simulink model "PIDControl"  (R2024b)
settings: Solver=VariableStepAuto  StartTime=0.0  StopTime=10.0  RelTol=1e-3
settings Model: Creator=mfussi  LastModifiedBy=mfussi

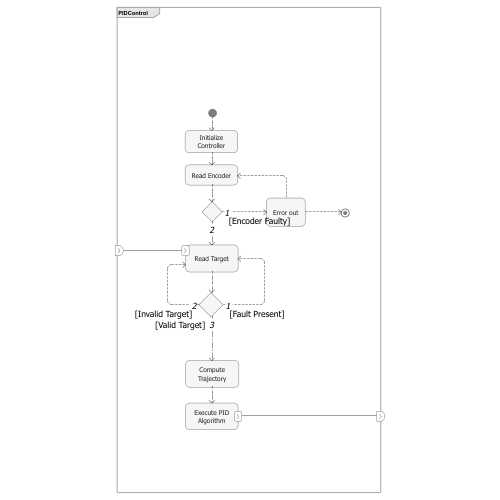
[thumbnail: Simulink's stored preview of the top-level diagram]
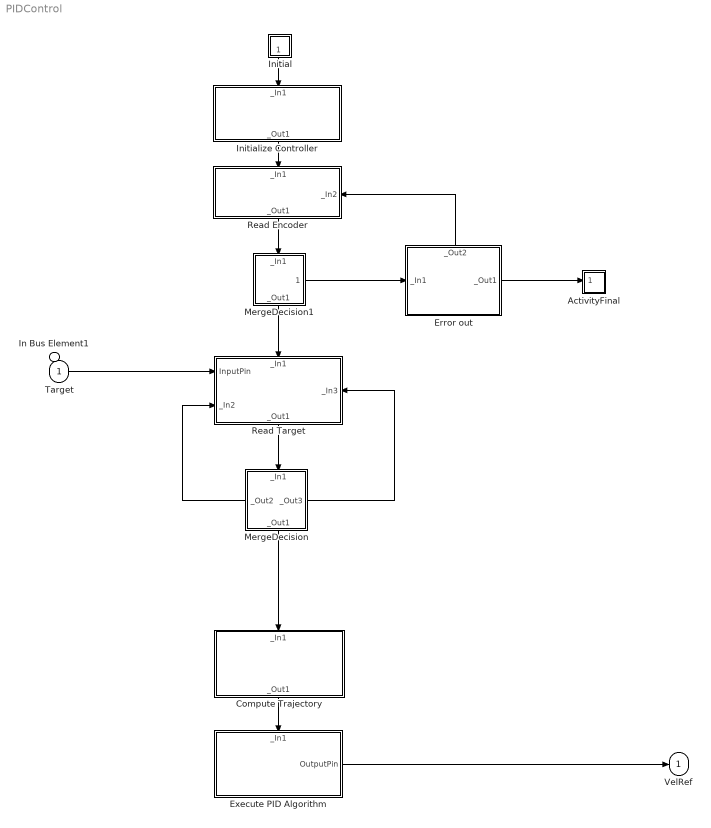
== system PIDControl ==
  Target : Inport
  In Bus Element1 : Inport  Port=2  PortName=Mode Selector
  ActivityFinal : Subsystem
      settings: CopyFcn=set_param(gcbh,'LinkStatus','none');  PortSchema="{\"entries\":[{\"content\":{\"sides\":[{\"content\":{\"connectorIds\":[\"In1\"]},\"type\":\"ConnectorPlacement.EquallySpacedRectSide\",\"uuid\":\"678327c4-9999-46ea-b1a4-4ad8eb3b1b3a\"},{\"content\":{\"side\":\"RIGHT\"},\"type\":\"ConnectorPlacement.EquallySpacedRectSide\",\"uuid\":\"7ffe71f3-976b-4666-94ba-13c7644f2cbe\"},{\"content\":{\"side\":\"TOP\"},\"type\":\"ConnectorPlacement.EquallySpacedRectSide\",\"uuid\":\"03885a3a-b599-465a-8063-ad719b644f55\"},{\"content\":{\"side\":\"BOTTOM\"},\"type\":\"ConnectorPlacement.EquallySpacedRectSide\",\"uuid\":\"d009bb3b-aa89-4ee7-8f41-c24160e2d423\"}]},\"type\":\"ConnectorPlacement.EquallySpacedConnector\",\"uuid\":\"2627a4b4-c689-4e44-af71-c1f35367d4c9\"}],\"packageUris\":[\"http://schema.mathworks.com/mf0/Connector/R2020b\"],\"version\":\"1.0\"}"
  Compute Trajectory : Subsystem
      settings: CopyFcn=set_param(gcbh,'LinkStatus','none');  PortSchema="{\"entries\":[{\"content\":{\"sides\":[{\"content\":{},\"type\":\"ConnectorPlacement.EquallySpacedRectSide\",\"uuid\":\"0e30ff93-cc66-4be0-9bd0-981231cc24fc\"},{\"content\":{\"side\":\"RIGHT\"},\"type\":\"ConnectorPlacement.EquallySpacedRectSide\",\"uuid\":\"7fcb7107-d79b-404e-9830-eb1616ed776d\"},{\"content\":{\"connectorIds\":[\"In1\"],\"side\":\"TOP\"},\"type\":\"ConnectorPlacement.EquallySpacedRectSide\",\"uuid\":\"d4d6ae97-3d3c-46b5-8a60-67bdf87a7c52\"},{\"content\":{\"connectorIds\":[\"Out1\"],\"side\":\"BOTTOM\"},\"type\":\"ConnectorPlacement.EquallySpacedRectSide\",\"uuid\":\"67ccb06d-41b1-4872-9b00-a9268e06f459\"}]},\"type\":\"ConnectorPlacement.EquallySpacedConnector\",\"uuid\":\"22b63578-781a-410c-8e5f-58d259414e27\"}],\"packageUris\":[\"http://schema.mathworks.com/mf0/Connector/R2020b\"],\"version\":\"1.0\"}"
  Error out : Subsystem
      settings: CopyFcn=set_param(gcbh,'LinkStatus','none');  PortSchema="{\"entries\":[{\"content\":{\"sides\":[{\"content\":{\"connectorIds\":[\"In1\"]},\"type\":\"ConnectorPlacement.EquallySpacedRectSide\",\"uuid\":\"0e30ff93-cc66-4be0-9bd0-981231cc24fc\"},{\"content\":{\"connectorIds\":[\"Out1\"],\"side\":\"RIGHT\"},\"type\":\"ConnectorPlacement.EquallySpacedRectSide\",\"uuid\":\"7fcb7107-d79b-404e-9830-eb1616ed776d\"},{\"content\":{\"connectorIds\":[\"Out2\"],\"side\":\"TOP\"},\"type\":\"ConnectorPlacement.EquallySpacedRectSide\",\"uuid\":\"d4d6ae97-3d3c-46b5-8a60-67bdf87a7c52\"}]},\"type\":\"ConnectorPlacement.EquallySpacedConnector\",\"uuid\":\"22b63578-781a-410c-8e5f-58d259414e27\"}],\"packageUris\":[\"http://schema.mathworks.com/mf0/Connector/R2020b\"],\"version\":\"1.0\"}"
  Execute PID Algorithm : Subsystem
      settings: CopyFcn=set_param(gcbh,'LinkStatus','none');  PortSchema="{\"entries\":[{\"content\":{\"sides\":[{\"content\":{},\"type\":\"ConnectorPlacement.EquallySpacedRectSide\",\"uuid\":\"0e30ff93-cc66-4be0-9bd0-981231cc24fc\"},{\"content\":{\"connectorIds\":[\"Out1\"],\"side\":\"RIGHT\"},\"type\":\"ConnectorPlacement.EquallySpacedRectSide\",\"uuid\":\"7fcb7107-d79b-404e-9830-eb1616ed776d\"},{\"content\":{\"connectorIds\":[\"In1\"],\"side\":\"TOP\"},\"type\":\"ConnectorPlacement.EquallySpacedRectSide\",\"uuid\":\"d4d6ae97-3d3c-46b5-8a60-67bdf87a7c52\"},{\"content\":{\"side\":\"BOTTOM\"},\"type\":\"ConnectorPlacement.EquallySpacedRectSide\",\"uuid\":\"6bb867f0-3dfa-4289-b556-b836133f11fd\"}]},\"type\":\"ConnectorPlacement.EquallySpacedConnector\",\"uuid\":\"22b63578-781a-410c-8e5f-58d259414e27\"}],\"packageUris\":[\"http://schema.mathworks.com/mf0/Connector/R2020b\"],\"version\":\"1.0\"}"
  Initial : Subsystem
      settings: CopyFcn=set_param(gcbh,'LinkStatus','none');  PortSchema="{\"entries\":[{\"content\":{\"sides\":[{\"content\":{},\"type\":\"ConnectorPlacement.EquallySpacedRectSide\",\"uuid\":\"0e30ff93-cc66-4be0-9bd0-981231cc24fc\"},{\"content\":{\"side\":\"RIGHT\"},\"type\":\"ConnectorPlacement.EquallySpacedRectSide\",\"uuid\":\"7fcb7107-d79b-404e-9830-eb1616ed776d\"},{\"content\":{\"side\":\"TOP\"},\"type\":\"ConnectorPlacement.EquallySpacedRectSide\",\"uuid\":\"d4d6ae97-3d3c-46b5-8a60-67bdf87a7c52\"},{\"content\":{\"connectorIds\":[\"Out1\"],\"side\":\"BOTTOM\"},\"type\":\"ConnectorPlacement.EquallySpacedRectSide\",\"uuid\":\"3d275148-0975-473b-a0a8-8b79500db052\"}]},\"type\":\"ConnectorPlacement.EquallySpacedConnector\",\"uuid\":\"22b63578-781a-410c-8e5f-58d259414e27\"}],\"packageUris\":[\"http://schema.mathworks.com/mf0/Connector/R2020b\"],\"version\":\"1.0\"}"
  Initialize Controller : Subsystem
      settings: CopyFcn=set_param(gcbh,'LinkStatus','none');  PortSchema="{\"entries\":[{\"content\":{\"sides\":[{\"content\":{},\"type\":\"ConnectorPlacement.EquallySpacedRectSide\",\"uuid\":\"0e30ff93-cc66-4be0-9bd0-981231cc24fc\"},{\"content\":{\"side\":\"RIGHT\"},\"type\":\"ConnectorPlacement.EquallySpacedRectSide\",\"uuid\":\"7fcb7107-d79b-404e-9830-eb1616ed776d\"},{\"content\":{\"connectorIds\":[\"In1\"],\"side\":\"TOP\"},\"type\":\"ConnectorPlacement.EquallySpacedRectSide\",\"uuid\":\"d4d6ae97-3d3c-46b5-8a60-67bdf87a7c52\"},{\"content\":{\"connectorIds\":[\"Out1\"],\"side\":\"BOTTOM\"},\"type\":\"ConnectorPlacement.EquallySpacedRectSide\",\"uuid\":\"d34c9b50-e751-481d-a5d8-0cc114e020a1\"}]},\"type\":\"ConnectorPlacement.EquallySpacedConnector\",\"uuid\":\"22b63578-781a-410c-8e5f-58d259414e27\"}],\"packageUris\":[\"http://schema.mathworks.com/mf0/Connector/R2020b\"],\"version\":\"1.0\"}"
  MergeDecision : Subsystem
      settings: CopyFcn=set_param(gcbh,'LinkStatus','none');  PortSchema="{\"entries\":[{\"content\":{\"sides\":[{\"content\":{\"connectorIds\":[\"Out2\"]},\"type\":\"ConnectorPlacement.EquallySpacedRectSide\",\"uuid\":\"0e30ff93-cc66-4be0-9bd0-981231cc24fc\"},{\"content\":{\"connectorIds\":[\"Out1\"],\"side\":\"RIGHT\"},\"type\":\"ConnectorPlacement.EquallySpacedRectSide\",\"uuid\":\"7fcb7107-d79b-404e-9830-eb1616ed776d\"},{\"content\":{\"connectorIds\":[\"In1\"],\"side\":\"TOP\"},\"type\":\"ConnectorPlacement.EquallySpacedRectSide\",\"uuid\":\"d4d6ae97-3d3c-46b5-8a60-67bdf87a7c52\"},{\"content\":{\"connectorIds\":[\"Out3\"],\"side\":\"BOTTOM\"},\"type\":\"ConnectorPlacement.EquallySpacedRectSide\",\"uuid\":\"cf938c80-5b4e-43e4-80fa-a183bc660f69\"}]},\"type\":\"ConnectorPlacement.EquallySpacedConnector\",\"uuid\":\"22b63578-781a-410c-8e5f-58d259414e27\"}],\"packageUris\":[\"http://schema.mathworks.com/mf0/Connector/R2020b\"],\"version\":\"1.0\"}"
  MergeDecision1 : Subsystem
      settings: CopyFcn=set_param(gcbh,'LinkStatus','none');  PortSchema="{\"entries\":[{\"content\":{\"sides\":[{\"content\":{},\"type\":\"ConnectorPlacement.EquallySpacedRectSide\",\"uuid\":\"0e30ff93-cc66-4be0-9bd0-981231cc24fc\"},{\"content\":{\"connectorIds\":[\"Out1\"],\"side\":\"RIGHT\"},\"type\":\"ConnectorPlacement.EquallySpacedRectSide\",\"uuid\":\"7fcb7107-d79b-404e-9830-eb1616ed776d\"},{\"content\":{\"connectorIds\":[\"In1\"],\"side\":\"TOP\"},\"type\":\"ConnectorPlacement.EquallySpacedRectSide\",\"uuid\":\"d4d6ae97-3d3c-46b5-8a60-67bdf87a7c52\"},{\"content\":{\"connectorIds\":[\"Out2\"],\"side\":\"BOTTOM\"},\"type\":\"ConnectorPlacement.EquallySpacedRectSide\",\"uuid\":\"0c32e27b-2b90-4df4-9155-f50c29ca6717\"}]},\"type\":\"ConnectorPlacement.EquallySpacedConnector\",\"uuid\":\"22b63578-781a-410c-8e5f-58d259414e27\"}],\"packageUris\":[\"http://schema.mathworks.com/mf0/Connector/R2020b\"],\"version\":\"1.0\"}"
  Read Encoder : Subsystem
      settings: CopyFcn=set_param(gcbh,'LinkStatus','none');  PortSchema="{\"entries\":[{\"content\":{\"sides\":[{\"content\":{},\"type\":\"ConnectorPlacement.EquallySpacedRectSide\",\"uuid\":\"0e30ff93-cc66-4be0-9bd0-981231cc24fc\"},{\"content\":{\"connectorIds\":[\"In1\"],\"side\":\"RIGHT\"},\"type\":\"ConnectorPlacement.EquallySpacedRectSide\",\"uuid\":\"7fcb7107-d79b-404e-9830-eb1616ed776d\"},{\"content\":{\"connectorIds\":[\"In2\"],\"side\":\"TOP\"},\"type\":\"ConnectorPlacement.EquallySpacedRectSide\",\"uuid\":\"d4d6ae97-3d3c-46b5-8a60-67bdf87a7c52\"},{\"content\":{\"connectorIds\":[\"Out1\"],\"side\":\"BOTTOM\"},\"type\":\"ConnectorPlacement.EquallySpacedRectSide\",\"uuid\":\"d34c9b50-e751-481d-a5d8-0cc114e020a1\"}]},\"type\":\"ConnectorPlacement.EquallySpacedConnector\",\"uuid\":\"22b63578-781a-410c-8e5f-58d259414e27\"}],\"packageUris\":[\"http://schema.mathworks.com/mf0/Connector/R2020b\"],\"version\":\"1.0\"}"
  Read Target : Subsystem
      settings: CopyFcn=set_param(gcbh,'LinkStatus','none');  PortSchema="{\"entries\":[{\"content\":{\"sides\":[{\"content\":{\"connectorIds\":[\"In1\",\"In3\"]},\"type\":\"ConnectorPlacement.EquallySpacedRectSide\",\"uuid\":\"0e30ff93-cc66-4be0-9bd0-981231cc24fc\"},{\"content\":{\"connectorIds\":[\"In2\"],\"side\":\"RIGHT\"},\"type\":\"ConnectorPlacement.EquallySpacedRectSide\",\"uuid\":\"7fcb7107-d79b-404e-9830-eb1616ed776d\"},{\"content\":{\"connectorIds\":[\"In4\"],\"side\":\"TOP\"},\"type\":\"ConnectorPlacement.EquallySpacedRectSide\",\"uuid\":\"d4d6ae97-3d3c-46b5-8a60-67bdf87a7c52\"},{\"content\":{\"connectorIds\":[\"Out1\"],\"side\":\"BOTTOM\"},\"type\":\"ConnectorPlacement.EquallySpacedRectSide\",\"uuid\":\"cfe19e5e-3578-4649-98cf-94940d25018d\"}]},\"type\":\"ConnectorPlacement.EquallySpacedConnector\",\"uuid\":\"22b63578-781a-410c-8e5f-58d259414e27\"}],\"packageUris\":[\"http://schema.mathworks.com/mf0/Connector/R2020b\"],\"version\":\"1.0\"}"
  VelRef : Outport
  wires:
  Initial/1(_Out1) -> Initialize Controller/1(_In1)
  Initialize Controller/1(_Out1) -> Read Encoder/2(_In1)
  Compute Trajectory/1(_Out1) -> Execute PID Algorithm/1(_In1)
  Read Target/1(_Out1) -> MergeDecision/1(_In1)
  MergeDecision/3(_Out1) -> Compute Trajectory/1(_In1)
  MergeDecision/2(_Out2) -> Read Target/3(_In2)
  MergeDecision/1(_Out3) -> Read Target/2(_In3)
  Read Encoder/1(_Out1) -> MergeDecision1/1(_In1)
  MergeDecision1/2(_Out1) -> Read Target/4(_In1)
  MergeDecision1/1(_Out2) -> Error out/1(_In1)
  Error out/2(_Out2) -> Read Encoder/1(_In2)
  Error out/1(_Out1) -> ActivityFinal/1(_In1)
  Target/1 -> Read Target/1(InputPin)
  Execute PID Algorithm/1(OutputPin) -> VelRef/1

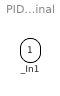
== system PIDControl/ActivityFinal ==
  _In1 : Inport

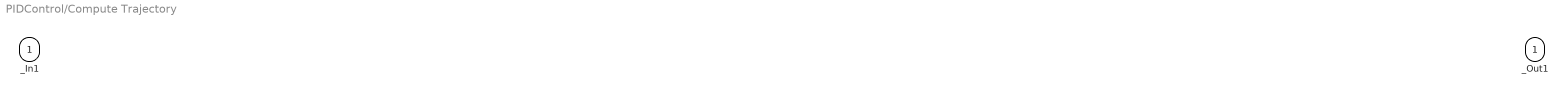
== system PIDControl/Compute Trajectory ==
  _In1 : Inport
  _Out1 : Outport

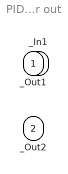
== system PIDControl/Error out ==
  _In1 : Inport
  _Out1 : Outport
  _Out2 : Outport  Port=2

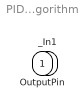
== system PIDControl/Execute PID Algorithm ==
  _In1 : Inport
  OutputPin : Outport  OutDataTypeStr=double  PortDimensions=1

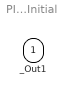
== system PIDControl/Initial ==
  _Out1 : Outport

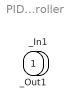
== system PIDControl/Initialize Controller ==
  _In1 : Inport
  _Out1 : Outport

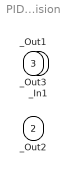
== system PIDControl/MergeDecision ==
  _In1 : Inport
  _Out3 : Outport
  _Out2 : Outport  Port=2
  _Out1 : Outport  Port=3

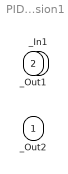
== system PIDControl/MergeDecision1 ==
  _In1 : Inport
  _Out2 : Outport
  _Out1 : Outport  Port=2

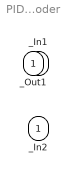
== system PIDControl/Read Encoder ==
  _In2 : Inport
  _In1 : Inport  Port=2
  _Out1 : Outport

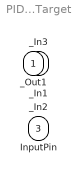
== system PIDControl/Read Target ==
  InputPin : Inport
  _In3 : Inport  Port=2
  _In2 : Inport  Port=3
  _In1 : Inport  Port=4
  _Out1 : Outport
